simulink model "QDVoltageSelectedDualConverter"  (R2026a)
settings: Solver=FixedStepDiscrete  StartTime=0  StopTime=0  FixedStep=1
InitFcn:
  | qdPackageRoot=fileparts(fileparts(get_param(bdroot,'FileName')));addpath(qdPackageRoot);setupQDVoltageSelectedDualConverter();initQDVoltageSelectedDualConverter(false);clear qdPackageRoot;
undefined symbols (not defined in the file): qdCCDdarkElectrons, qdCommonOutputWavelength_nm, qdIncidentSpectrum, qdInGaAsDetectorGain_ePerPhoton, qdSiDetectorGain_ePerPhoton, qdSpectrometerResponse, qdUpToCommonMatrix, qdUVIncidentSpectrum
Description:
  | Attached dual-path quantum-dot conversion system: powered SWIR-to-visible up-conversion or passive electronically selected UV-to-visible/NIR down-conversion, with detector and computation.
settings Model: Creator=jyohtiprakash  LastModifiedBy=jyohtiprakash

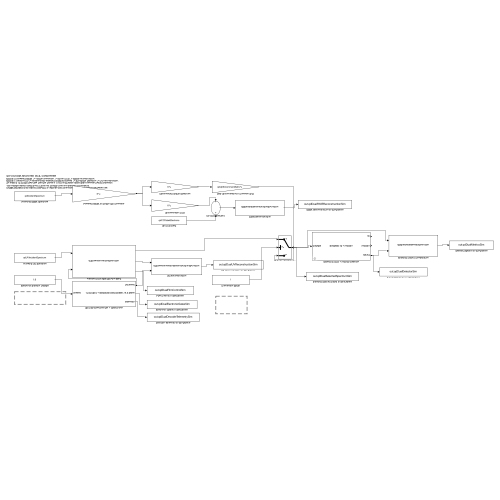
[thumbnail: Simulink's stored preview of the top-level diagram]
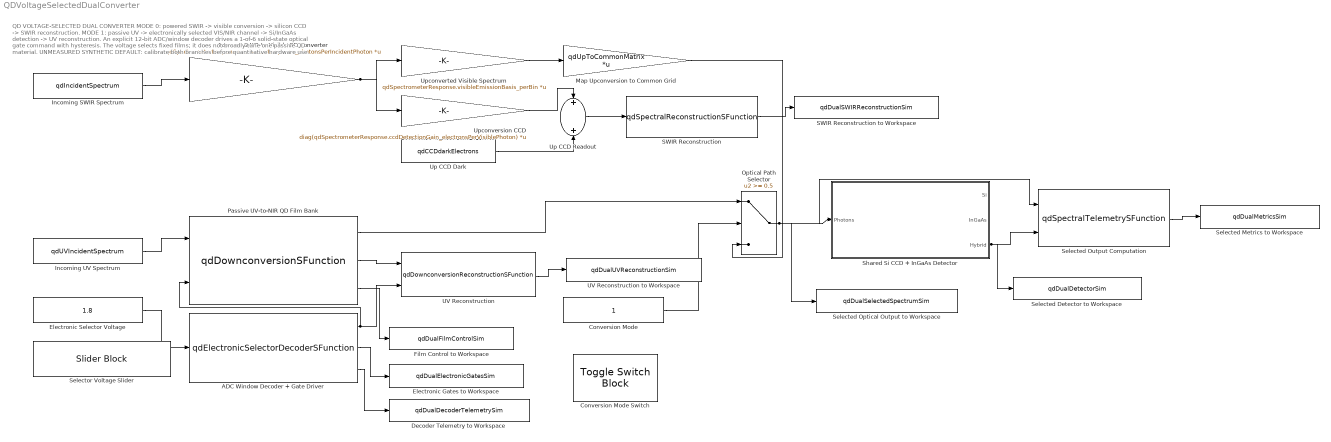
== system QDVoltageSelectedDualConverter ==
  note: QD VOLTAGE-SELECTED DUAL CONVERTER
      | MODE 0: powered SWIR -> visible conversion -> silicon CCD -> SWIR reconstruction.
      | MODE 1: passive UV -> electronically selected VIS/NIR channel -> Si/InGaAs detection -> UV reconstruction.
      | An explicit 12-bit ADC/window decoder drives a 1-of-6 solid-state optical gate command with hysteresis.
      | The voltage selects fixed films; it does not broadly tune one passive QD material.
      | UNMEASURED SYNTHETIC DEFAULT: calibrate both branches before quantitative hardware use.
  ADC Window Decoder + Gate Driver : M-S-Function  FunctionName=qdElectronicSelectorDecoderSFunction
      mask help: Electronic selector: ADC quantization, voltage-window decoding, comparator hysteresis, and one-hot optical-gate command.
      mask Display:
      | disp('12-bit ADC + WINDOW DECODER');
      | port_label('input',1,'Vselect');
      | port_label('output',1,'Vchannel');
      | port_label('output',2,'1-of-6 gates');
      | port_label('output',3,'telemetry');
  Conversion Mode : Constant
  Conversion Mode Switch : ToggleSwitchBlock
  Decoder Telemetry to Workspace : ToWorkspace  VariableName=qdDualDecoderTelemetrySim  SaveFormat=Structure With Time  SampleTime=-1
  Electronic Gates to Workspace : ToWorkspace  VariableName=qdDualElectronicGatesSim  SaveFormat=Structure With Time  SampleTime=-1
  Electronic Selector Voltage : Constant  Value=1.8
  Film Control to Workspace : ToWorkspace  VariableName=qdDualFilmControlSim  SaveFormat=Structure With Time  SampleTime=-1
  Incoming SWIR Spectrum : Constant  Value=qdIncidentSpectrum
  Incoming UV Spectrum : Constant  Value=qdUVIncidentSpectrum
  Map Upconversion to Common Grid : Gain  Gain=qdUpToCommonMatrix  Multiplication=Matrix(K*u)
  Optical Path Selector : Switch  Threshold=0.5  SaturateOnIntegerOverflow=off  InputSameDT=off
  Passive UV-to-NIR QD Film Bank : M-S-Function  FunctionName=qdDownconversionSFunction
  Powered SWIR-to-Visible QD Converter : Gain  Gain=qdSpectrometerResponse.converterResponse_photonsPerIncidentPhoton  Multiplication=Matrix(K*u)
  SWIR Reconstruction : M-S-Function  FunctionName=qdSpectralReconstructionSFunction
  SWIR Reconstruction to Workspace : ToWorkspace  VariableName=qdDualSWIRReconstructionSim  SaveFormat=Structure With Time  SampleTime=-1
  Selected Detector to Workspace : ToWorkspace  VariableName=qdDualDetectorSim  SaveFormat=Structure With Time  SampleTime=-1
  Selected Metrics to Workspace : ToWorkspace  VariableName=qdDualMetricsSim  SaveFormat=Structure With Time  SampleTime=-1
  Selected Optical Output to Workspace : ToWorkspace  VariableName=qdDualSelectedSpectrumSim  SaveFormat=Structure With Time  SampleTime=-1
  Selected Output Computation : M-S-Function  FunctionName=qdSpectralTelemetrySFunction
  Selector Voltage Slider : SliderBlock  ScaleMin=0.29999999999999999  ScaleMax=2.7999999999999998  TickInterval=0.49999999999999978
  Shared Si CCD + InGaAs Detector : Subsystem
      mask help: Dichroic split between a silicon CCD and an InGaAs array so the combined output grid is not limited by silicon cutoff.
      mask Display:
      | disp('SHARED Si + InGaAs');
      | port_label('input',1,'VIS/NIR');
      | port_label('output',1,'Si');
      | port_label('output',2,'InGaAs');
      | port_label('output',3,'hybrid');
  UV Reconstruction : M-S-Function  FunctionName=qdDownconversionReconstructionSFunction
  UV Reconstruction to Workspace : ToWorkspace  VariableName=qdDualUVReconstructionSim  SaveFormat=Structure With Time  SampleTime=-1
  Up CCD Dark : Constant  Value=qdCCDdarkElectrons
  Up CCD Readout : Sum
  Upconversion CCD : Gain  Gain=diag(qdSpectrometerResponse.ccdDetectionGain_electronsPerVisiblePhoton)  Multiplication=Matrix(K*u)
  Upconverted Visible Spectrum : Gain  Gain=qdSpectrometerResponse.visibleEmissionBasis_perBin  Multiplication=Matrix(K*u)
  wires:
  Incoming SWIR Spectrum/1 -> Powered SWIR-to-Visible QD Converter/1
  Powered SWIR-to-Visible QD Converter/1 -> Upconverted Visible Spectrum/1, Upconversion CCD/1
  Upconverted Visible Spectrum/1 -> Map Upconversion to Common Grid/1
  Upconversion CCD/1 -> Up CCD Readout/1
  Up CCD Dark/1 -> Up CCD Readout/2
  Up CCD Readout/1 -> SWIR Reconstruction/1
  Electronic Selector Voltage/1 -> ADC Window Decoder + Gate Driver/1
  Incoming UV Spectrum/1 -> Passive UV-to-NIR QD Film Bank/1
  ADC Window Decoder + Gate Driver/1 -> Passive UV-to-NIR QD Film Bank/2, UV Reconstruction/2
  Passive UV-to-NIR QD Film Bank/2 -> UV Reconstruction/1
  Passive UV-to-NIR QD Film Bank/1 -> Optical Path Selector/1
  Conversion Mode/1 -> Optical Path Selector/2
  Map Upconversion to Common Grid/1 -> Optical Path Selector/3
  Optical Path Selector/1 -> Shared Si CCD + InGaAs Detector/1(Photons), Selected Output Computation/1, Selected Optical Output to Workspace/1
  Shared Si CCD + InGaAs Detector/3(Hybrid) -> Selected Output Computation/2, Selected Detector to Workspace/1
  SWIR Reconstruction/1 -> SWIR Reconstruction to Workspace/1
  UV Reconstruction/1 -> UV Reconstruction to Workspace/1
  Passive UV-to-NIR QD Film Bank/3 -> Film Control to Workspace/1
  ADC Window Decoder + Gate Driver/2 -> Electronic Gates to Workspace/1
  ADC Window Decoder + Gate Driver/3 -> Decoder Telemetry to Workspace/1
  Selected Output Computation/1 -> Selected Metrics to Workspace/1

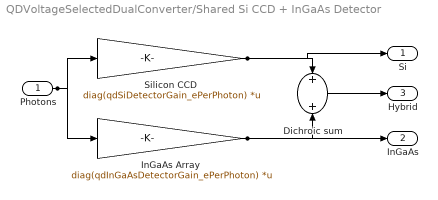
== system QDVoltageSelectedDualConverter/Shared Si CCD + InGaAs Detector ==
  Photons : Inport  PortDimensions=numel(qdCommonOutputWavelength_nm)
  Dichroic sum : Sum
  InGaAs Array : Gain  Gain=diag(qdInGaAsDetectorGain_ePerPhoton)  Multiplication=Matrix(K*u)
  Silicon CCD : Gain  Gain=diag(qdSiDetectorGain_ePerPhoton)  Multiplication=Matrix(K*u)
  Si : Outport  PortDimensions=numel(qdCommonOutputWavelength_nm)
  InGaAs : Outport  Port=2  PortDimensions=numel(qdCommonOutputWavelength_nm)
  Hybrid : Outport  Port=3  PortDimensions=numel(qdCommonOutputWavelength_nm)
  wires:
  Photons/1 -> Silicon CCD/1, InGaAs Array/1
  Silicon CCD/1 -> Dichroic sum/1, Si/1
  InGaAs Array/1 -> Dichroic sum/2, InGaAs/1
  Dichroic sum/1 -> Hybrid/1
